simulink model "Dual_EV_Charger_baseline"  (R2025b)
settings: Solver=ode23t  StartTime=0.0  StopTime=0.5  RelTol=1e-3
libraries: fl_lib x98, nesl_utility x24, ee_lib x6, slpidlib x4, batteryecm_lib x4, eePwmGenerator x2
(part 3 of 3)

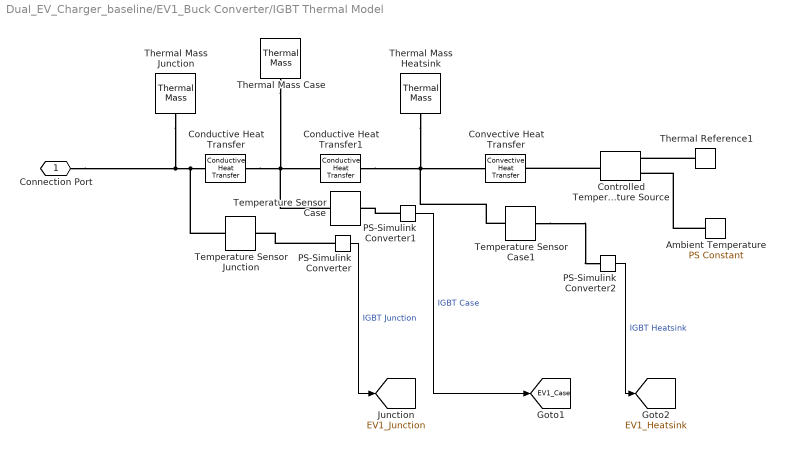
== system Dual_EV_Charger_baseline/EV1_Buck Converter/IGBT Thermal Model ==
  Ambient Temperature : fl_lib/Physical Signals/Sources/PS Constant  constant=298.15
  Conductive Heat Transfer : fl_lib/Thermal/Thermal Elements/Conductive Heat Transfer  thermal_type=foundation.enum.ConstantVariableTabulated.Constant  wall_geometry=foundation.enum.ConductionWallGeometry.Planar  area=5 m^2  thickness=360 m  d_in=0.05 m  d_out=0.1 m  L=1 m  th_cond_min=10 W/(K*m)  th_cond=150 W/(K*m)  th_cond_TLU=[413, 401, 392, 383, 371, 357, 342] W/(K*m)  temp_TLU=[200, 273, 400, 600, 800, 1000, 1200] K  T_specify=off  T_priority=None  T=0 K  T_nominal_specify=off  T_nominal_value=1  T_nominal_unit=K  Q_specify=off  Q_priority=None  Q=0 W  Q_nominal_specify=off  Q_nominal_value=1  Q_nominal_unit=W
  Conductive Heat Transfer1 : fl_lib/Thermal/Thermal Elements/Conductive Heat Transfer  thermal_type=foundation.enum.ConstantVariableTabulated.Constant  wall_geometry=foundation.enum.ConductionWallGeometry.Planar  area=14 m^2  thickness=0.1 m  d_in=0.05 m  d_out=0.1 m  L=1 m  th_cond_min=10 W/(K*m)  th_cond=3 W/(K*m)  th_cond_TLU=[413, 401, 392, 383, 371, 357, 342] W/(K*m)  temp_TLU=[200, 273, 400, 600, 800, 1000, 1200] K  T_specify=off  T_priority=None  T=0 K  T_nominal_specify=off  T_nominal_value=1  T_nominal_unit=K  Q_specify=off  Q_priority=None  Q=0 W  Q_nominal_specify=off  Q_nominal_value=1  Q_nominal_unit=W
  Controlled Temperature Source : fl_lib/Thermal/Thermal Sources/Controlled Temperature Source
  Convective Heat Transfer : fl_lib/Thermal/Thermal Elements/Convective Heat Transfer  thermal_type=foundation.enum.constant_variable.constant  area=40 m^2  heat_tr_coeff=20 W/(K*m^2)  min_heat_tr_coeff=1e-3 W/(K*m^2)  T_specify=off  T_priority=None  T=0 K  T_nominal_specify=off  T_nominal_value=1  T_nominal_unit=K  Q_specify=off  Q_priority=None  Q=0 W  Q_nominal_specify=off  Q_nominal_value=1  Q_nominal_unit=W
  PS-Simulink Converter : nesl_utility/PS-Simulink Converter  PhysicalDomain=network_engine_domain  SubClassName=ps_output  LeftPortType=input  RightPortType=output  PseudoPeriodic=off  Frequencies=[]  VectorFormat=inherit  Unit=inherit  AffineConversion=off
  PS-Simulink Converter1 : nesl_utility/PS-Simulink Converter  PhysicalDomain=network_engine_domain  SubClassName=ps_output  LeftPortType=input  RightPortType=output  PseudoPeriodic=off  Frequencies=[]  VectorFormat=inherit  Unit=inherit  AffineConversion=off
  PS-Simulink Converter2 : nesl_utility/PS-Simulink Converter  PhysicalDomain=network_engine_domain  SubClassName=ps_output  LeftPortType=input  RightPortType=output  PseudoPeriodic=off  Frequencies=[]  VectorFormat=inherit  Unit=inherit  AffineConversion=off
  Temperature Sensor Case : fl_lib/Thermal/Thermal Sensors/Temperature Sensor  temperature_measure=foundation.enum.MeasurementReference.absolute
      settings: InternalSimscapePortConfiguration="{\"Bottom\":[],\"Left\":[{\"id\":\"A\",\"label\":\"A\",\"type\":\"foundation.thermal.thermal\"}],\"Right\":[{\"id\":\"T\",\"label\":\"T\",\"type\":\"output\"}],\"Top\":[]}"
  Temperature Sensor Case1 : fl_lib/Thermal/Thermal Sensors/Temperature Sensor  temperature_measure=foundation.enum.MeasurementReference.absolute
      settings: InternalSimscapePortConfiguration="{\"Bottom\":[],\"Left\":[{\"id\":\"A\",\"label\":\"A\",\"type\":\"foundation.thermal.thermal\"}],\"Right\":[{\"id\":\"T\",\"label\":\"T\",\"type\":\"output\"}],\"Top\":[]}"
  Temperature Sensor Junction : fl_lib/Thermal/Thermal Sensors/Temperature Sensor  temperature_measure=foundation.enum.MeasurementReference.absolute
      settings: InternalSimscapePortConfiguration="{\"Bottom\":[],\"Left\":[{\"id\":\"A\",\"label\":\"A\",\"type\":\"foundation.thermal.thermal\"}],\"Right\":[{\"id\":\"T\",\"label\":\"T\",\"type\":\"output\"}],\"Top\":[]}"
  Thermal Mass Case : fl_lib/Thermal/Thermal Elements/Thermal Mass  mass_type=foundation.enum.constant_variable.constant  mass=0.02 kg  sp_heat=385 J/(K*kg)  mass_min=1e-6 kg  num_ports=foundation.enum.numPorts2.one  m_specify=off  m_priority=High  m=1 kg  m_nominal_specify=off  m_nominal_value=1  m_nominal_unit=kg  T_specify=on  T_priority=High  T=298.15 K  T_nominal_specify=off  T_nominal_value=1  T_nominal_unit=K  Q_specify=off  Q_priority=None  Q=0 W  Q_nominal_specify=off  Q_nominal_value=1  Q_nominal_unit=W
  Thermal Mass Heatsink : fl_lib/Thermal/Thermal Elements/Thermal Mass  mass_type=foundation.enum.constant_variable.constant  mass=0.2 kg  sp_heat=900 J/(K*kg)  mass_min=1e-6 kg  num_ports=foundation.enum.numPorts2.one  m_specify=off  m_priority=High  m=1 kg  m_nominal_specify=off  m_nominal_value=1  m_nominal_unit=kg  T_specify=on  T_priority=High  T=298.15 K  T_nominal_specify=off  T_nominal_value=1  T_nominal_unit=K  Q_specify=off  Q_priority=None  Q=0 W  Q_nominal_specify=off  Q_nominal_value=1  Q_nominal_unit=W
  Thermal Mass Junction : fl_lib/Thermal/Thermal Elements/Thermal Mass  mass_type=foundation.enum.constant_variable.constant  mass=0.001 kg  sp_heat=700 J/(K*kg)  mass_min=1e-6 kg  num_ports=foundation.enum.numPorts2.one  m_specify=off  m_priority=High  m=1 kg  m_nominal_specify=off  m_nominal_value=1  m_nominal_unit=kg  T_specify=on  T_priority=High  T="298.15  K"  T_nominal_specify=off  T_nominal_value=1  T_nominal_unit=K  Q_specify=off  Q_priority=None  Q=0 W  Q_nominal_specify=off  Q_nominal_value=1  Q_nominal_unit=W
  Thermal Reference1 : fl_lib/Thermal/Thermal Elements/Thermal Reference
  Connection Port : PMIOPort  Side=Left
  tag scope: EV1_Case=global, EV1_Heatsink=global, EV1_Junction=global
  wires:
  PS-Simulink Converter/1 -> [EV1_Junction]  "IGBT Junction"
  PS-Simulink Converter1/1 -> [EV1_Case]  "IGBT Case"
  PS-Simulink Converter2/1 -> [EV1_Heatsink]  "IGBT Heatsink"
  connections:
  Conductive Heat Transfer1/RConn1 -- Temperature Sensor Case1/LConn1 -- Thermal Mass Heatsink/LConn1 -- Convective Heat Transfer/LConn1
  Conductive Heat Transfer/RConn1 -- Thermal Mass Case/LConn1 -- Temperature Sensor Case/LConn1 -- Conductive Heat Transfer1/LConn1
  Connection Port/RConn1 -- Thermal Mass Junction/LConn1 -- Temperature Sensor Junction/LConn1 -- Conductive Heat Transfer/LConn1
  Controlled Temperature Source/LConn1 -- Convective Heat Transfer/RConn1
  Thermal Reference1/LConn1 -- Controlled Temperature Source/RConn2
  PS-Simulink Converter/LConn1 -- Temperature Sensor Junction/RConn1
  Ambient Temperature/RConn1 -- Controlled Temperature Source/RConn1
  PS-Simulink Converter1/LConn1 -- Temperature Sensor Case/RConn1
  Temperature Sensor Case1/RConn1 -- PS-Simulink Converter2/LConn1

== system Dual_EV_Charger_baseline/EV1_Plant//EV Battery/EV Battery Thermal Model ==
  Ambient Temperature1 : fl_lib/Physical Signals/Sources/PS Constant  constant=292.15
  Controlled Temperature Source : fl_lib/Thermal/Thermal Sources/Controlled Temperature Source
  Convective Heat Transfer : fl_lib/Thermal/Thermal Elements/Convective Heat Transfer  thermal_type=foundation.enum.constant_variable.constant  area=1e-4 m^2  heat_tr_coeff=20 W/(K*m^2)  min_heat_tr_coeff=1e-3 W/(K*m^2)  T_specify=off  T_priority=None  T=0 K  T_nominal_specify=off  T_nominal_value=1  T_nominal_unit=K  Q_specify=off  Q_priority=None  Q=0 W  Q_nominal_specify=off  Q_nominal_value=1  Q_nominal_unit=W
  PS-Simulink Converter : nesl_utility/PS-Simulink Converter  PhysicalDomain=network_engine_domain  SubClassName=ps_output  LeftPortType=input  RightPortType=output  PseudoPeriodic=off  Frequencies=[]  VectorFormat=inherit  Unit=inherit  AffineConversion=off
  Temperature Sensor : fl_lib/Thermal/Thermal Sensors/Temperature Sensor  temperature_measure=foundation.enum.MeasurementReference.difference
  Thermal Reference : fl_lib/Thermal/Thermal Elements/Thermal Reference
  Thermal Port : PMIOPort  Side=Left
  tag scope: EV1_Tempertaure=global
  wires:
  PS-Simulink Converter/1 -> [EV1_Tempertaure]
  connections:
  Temperature Sensor/LConn1 -- Thermal Port/RConn1 -- Convective Heat Transfer/LConn1
  Convective Heat Transfer/RConn1 -- Controlled Temperature Source/LConn1
  Temperature Sensor/RConn1 -- Controlled Temperature Source/RConn2 -- Thermal Reference/LConn1
  Controlled Temperature Source/RConn1 -- Ambient Temperature1/RConn1
  PS-Simulink Converter/LConn1 -- Temperature Sensor/RConn2

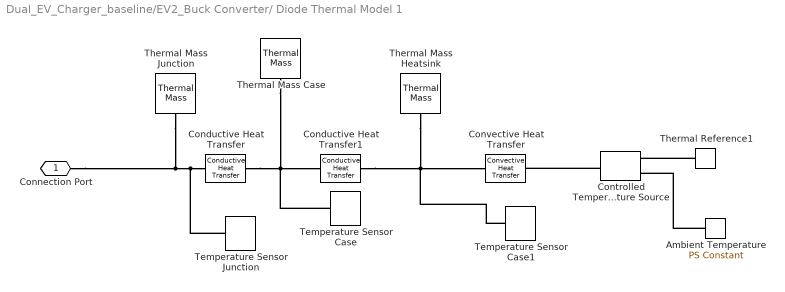
== system Dual_EV_Charger_baseline/EV2_Buck Converter/ Diode Thermal Model 1 ==
  Ambient Temperature : fl_lib/Physical Signals/Sources/PS Constant  constant=298.15
  Conductive Heat Transfer : fl_lib/Thermal/Thermal Elements/Conductive Heat Transfer  thermal_type=foundation.enum.ConstantVariableTabulated.Constant  wall_geometry=foundation.enum.ConductionWallGeometry.Planar  area=5 m^2  thickness=360 m  d_in=0.05 m  d_out=0.1 m  L=1 m  th_cond_min=10 W/(K*m)  th_cond=150 W/(K*m)  th_cond_TLU=[413, 401, 392, 383, 371, 357, 342] W/(K*m)  temp_TLU=[200, 273, 400, 600, 800, 1000, 1200] K  T_specify=off  T_priority=None  T=0 K  T_nominal_specify=off  T_nominal_value=1  T_nominal_unit=K  Q_specify=off  Q_priority=None  Q=0 W  Q_nominal_specify=off  Q_nominal_value=1  Q_nominal_unit=W
  Conductive Heat Transfer1 : fl_lib/Thermal/Thermal Elements/Conductive Heat Transfer  thermal_type=foundation.enum.ConstantVariableTabulated.Constant  wall_geometry=foundation.enum.ConductionWallGeometry.Planar  area=14 m^2  thickness=0.1 m  d_in=0.05 m  d_out=0.1 m  L=1 m  th_cond_min=10 W/(K*m)  th_cond=3 W/(K*m)  th_cond_TLU=[413, 401, 392, 383, 371, 357, 342] W/(K*m)  temp_TLU=[200, 273, 400, 600, 800, 1000, 1200] K  T_specify=off  T_priority=None  T=0 K  T_nominal_specify=off  T_nominal_value=1  T_nominal_unit=K  Q_specify=off  Q_priority=None  Q=0 W  Q_nominal_specify=off  Q_nominal_value=1  Q_nominal_unit=W
  Controlled Temperature Source : fl_lib/Thermal/Thermal Sources/Controlled Temperature Source
  Convective Heat Transfer : fl_lib/Thermal/Thermal Elements/Convective Heat Transfer  thermal_type=foundation.enum.constant_variable.constant  area=40 m^2  heat_tr_coeff=20 W/(K*m^2)  min_heat_tr_coeff=1e-3 W/(K*m^2)  T_specify=off  T_priority=None  T=0 K  T_nominal_specify=off  T_nominal_value=1  T_nominal_unit=K  Q_specify=off  Q_priority=None  Q=0 W  Q_nominal_specify=off  Q_nominal_value=1  Q_nominal_unit=W
  Temperature Sensor Case : fl_lib/Thermal/Thermal Sensors/Temperature Sensor  temperature_measure=foundation.enum.MeasurementReference.absolute
      settings: InternalSimscapePortConfiguration="{\"Bottom\":[],\"Left\":[{\"id\":\"A\",\"label\":\"A\",\"type\":\"foundation.thermal.thermal\"}],\"Right\":[{\"id\":\"T\",\"label\":\"T\",\"type\":\"output\"}],\"Top\":[]}"
  Temperature Sensor Case1 : fl_lib/Thermal/Thermal Sensors/Temperature Sensor  temperature_measure=foundation.enum.MeasurementReference.absolute
      settings: InternalSimscapePortConfiguration="{\"Bottom\":[],\"Left\":[{\"id\":\"A\",\"label\":\"A\",\"type\":\"foundation.thermal.thermal\"}],\"Right\":[{\"id\":\"T\",\"label\":\"T\",\"type\":\"output\"}],\"Top\":[]}"
  Temperature Sensor Junction : fl_lib/Thermal/Thermal Sensors/Temperature Sensor  temperature_measure=foundation.enum.MeasurementReference.absolute
      settings: InternalSimscapePortConfiguration="{\"Bottom\":[],\"Left\":[{\"id\":\"A\",\"label\":\"A\",\"type\":\"foundation.thermal.thermal\"}],\"Right\":[{\"id\":\"T\",\"label\":\"T\",\"type\":\"output\"}],\"Top\":[]}"
  Thermal Mass Case : fl_lib/Thermal/Thermal Elements/Thermal Mass  mass_type=foundation.enum.constant_variable.constant  mass=0.02 kg  sp_heat=385 J/(K*kg)  mass_min=1e-6 kg  num_ports=foundation.enum.numPorts2.one  m_specify=off  m_priority=High  m=1 kg  m_nominal_specify=off  m_nominal_value=1  m_nominal_unit=kg  T_specify=on  T_priority=High  T=298.15 K  T_nominal_specify=off  T_nominal_value=1  T_nominal_unit=K  Q_specify=off  Q_priority=None  Q=0 W  Q_nominal_specify=off  Q_nominal_value=1  Q_nominal_unit=W
  Thermal Mass Heatsink : fl_lib/Thermal/Thermal Elements/Thermal Mass  mass_type=foundation.enum.constant_variable.constant  mass=0.2 kg  sp_heat=900 J/(K*kg)  mass_min=1e-6 kg  num_ports=foundation.enum.numPorts2.one  m_specify=off  m_priority=High  m=1 kg  m_nominal_specify=off  m_nominal_value=1  m_nominal_unit=kg  T_specify=on  T_priority=High  T=298.15 K  T_nominal_specify=off  T_nominal_value=1  T_nominal_unit=K  Q_specify=off  Q_priority=None  Q=0 W  Q_nominal_specify=off  Q_nominal_value=1  Q_nominal_unit=W
  Thermal Mass Junction : fl_lib/Thermal/Thermal Elements/Thermal Mass  mass_type=foundation.enum.constant_variable.constant  mass=0.001 kg  sp_heat=700 J/(K*kg)  mass_min=1e-6 kg  num_ports=foundation.enum.numPorts2.one  m_specify=off  m_priority=High  m=1 kg  m_nominal_specify=off  m_nominal_value=1  m_nominal_unit=kg  T_specify=on  T_priority=High  T="298.15  K"  T_nominal_specify=off  T_nominal_value=1  T_nominal_unit=K  Q_specify=off  Q_priority=None  Q=0 W  Q_nominal_specify=off  Q_nominal_value=1  Q_nominal_unit=W
  Thermal Reference1 : fl_lib/Thermal/Thermal Elements/Thermal Reference
  Connection Port : PMIOPort  Side=Left
  connections:
  Conductive Heat Transfer1/RConn1 -- Thermal Mass Heatsink/LConn1 -- Convective Heat Transfer/LConn1 -- Temperature Sensor Case1/LConn1
  Thermal Mass Case/LConn1 -- Conductive Heat Transfer/RConn1 -- Conductive Heat Transfer1/LConn1 -- Temperature Sensor Case/LConn1
  Thermal Mass Junction/LConn1 -- Temperature Sensor Junction/LConn1 -- Conductive Heat Transfer/LConn1 -- Connection Port/RConn1
  Controlled Temperature Source/LConn1 -- Convective Heat Transfer/RConn1
  Thermal Reference1/LConn1 -- Controlled Temperature Source/RConn2
  Ambient Temperature/RConn1 -- Controlled Temperature Source/RConn1

== system Dual_EV_Charger_baseline/EV2_Buck Converter/ Diode Thermal Model 2 ==
  Ambient Temperature : fl_lib/Physical Signals/Sources/PS Constant  constant=298.15
  Conductive Heat Transfer : fl_lib/Thermal/Thermal Elements/Conductive Heat Transfer  thermal_type=foundation.enum.ConstantVariableTabulated.Constant  wall_geometry=foundation.enum.ConductionWallGeometry.Planar  area=5 m^2  thickness=360 m  d_in=0.05 m  d_out=0.1 m  L=1 m  th_cond_min=10 W/(K*m)  th_cond=150 W/(K*m)  th_cond_TLU=[413, 401, 392, 383, 371, 357, 342] W/(K*m)  temp_TLU=[200, 273, 400, 600, 800, 1000, 1200] K  T_specify=off  T_priority=None  T=0 K  T_nominal_specify=off  T_nominal_value=1  T_nominal_unit=K  Q_specify=off  Q_priority=None  Q=0 W  Q_nominal_specify=off  Q_nominal_value=1  Q_nominal_unit=W
  Conductive Heat Transfer1 : fl_lib/Thermal/Thermal Elements/Conductive Heat Transfer  thermal_type=foundation.enum.ConstantVariableTabulated.Constant  wall_geometry=foundation.enum.ConductionWallGeometry.Planar  area=14 m^2  thickness=0.1 m  d_in=0.05 m  d_out=0.1 m  L=1 m  th_cond_min=10 W/(K*m)  th_cond=3 W/(K*m)  th_cond_TLU=[413, 401, 392, 383, 371, 357, 342] W/(K*m)  temp_TLU=[200, 273, 400, 600, 800, 1000, 1200] K  T_specify=off  T_priority=None  T=0 K  T_nominal_specify=off  T_nominal_value=1  T_nominal_unit=K  Q_specify=off  Q_priority=None  Q=0 W  Q_nominal_specify=off  Q_nominal_value=1  Q_nominal_unit=W
  Controlled Temperature Source : fl_lib/Thermal/Thermal Sources/Controlled Temperature Source
  Convective Heat Transfer : fl_lib/Thermal/Thermal Elements/Convective Heat Transfer  thermal_type=foundation.enum.constant_variable.constant  area=40 m^2  heat_tr_coeff=20 W/(K*m^2)  min_heat_tr_coeff=1e-3 W/(K*m^2)  T_specify=off  T_priority=None  T=0 K  T_nominal_specify=off  T_nominal_value=1  T_nominal_unit=K  Q_specify=off  Q_priority=None  Q=0 W  Q_nominal_specify=off  Q_nominal_value=1  Q_nominal_unit=W
  EV2_Temperature Sensor Case : fl_lib/Thermal/Thermal Sensors/Temperature Sensor  temperature_measure=foundation.enum.MeasurementReference.absolute
      settings: InternalSimscapePortConfiguration="{\"Bottom\":[],\"Left\":[{\"id\":\"A\",\"label\":\"A\",\"type\":\"foundation.thermal.thermal\"}],\"Right\":[{\"id\":\"T\",\"label\":\"T\",\"type\":\"output\"}],\"Top\":[]}"
  EV2_Temperature Sensor Case1 : fl_lib/Thermal/Thermal Sensors/Temperature Sensor  temperature_measure=foundation.enum.MeasurementReference.absolute
      settings: InternalSimscapePortConfiguration="{\"Bottom\":[],\"Left\":[{\"id\":\"A\",\"label\":\"A\",\"type\":\"foundation.thermal.thermal\"}],\"Right\":[{\"id\":\"T\",\"label\":\"T\",\"type\":\"output\"}],\"Top\":[]}"
  EV2_Temperature Sensor Junction : fl_lib/Thermal/Thermal Sensors/Temperature Sensor  temperature_measure=foundation.enum.MeasurementReference.absolute
      settings: InternalSimscapePortConfiguration="{\"Bottom\":[],\"Left\":[{\"id\":\"A\",\"label\":\"A\",\"type\":\"foundation.thermal.thermal\"}],\"Right\":[{\"id\":\"T\",\"label\":\"T\",\"type\":\"output\"}],\"Top\":[]}"
  Thermal Mass Case : fl_lib/Thermal/Thermal Elements/Thermal Mass  mass_type=foundation.enum.constant_variable.constant  mass=0.02 kg  sp_heat=385 J/(K*kg)  mass_min=1e-6 kg  num_ports=foundation.enum.numPorts2.one  m_specify=off  m_priority=High  m=1 kg  m_nominal_specify=off  m_nominal_value=1  m_nominal_unit=kg  T_specify=on  T_priority=High  T=298.15 K  T_nominal_specify=off  T_nominal_value=1  T_nominal_unit=K  Q_specify=off  Q_priority=None  Q=0 W  Q_nominal_specify=off  Q_nominal_value=1  Q_nominal_unit=W
  Thermal Mass Heatsink : fl_lib/Thermal/Thermal Elements/Thermal Mass  mass_type=foundation.enum.constant_variable.constant  mass=0.2 kg  sp_heat=900 J/(K*kg)  mass_min=1e-6 kg  num_ports=foundation.enum.numPorts2.one  m_specify=off  m_priority=High  m=1 kg  m_nominal_specify=off  m_nominal_value=1  m_nominal_unit=kg  T_specify=on  T_priority=High  T=298.15 K  T_nominal_specify=off  T_nominal_value=1  T_nominal_unit=K  Q_specify=off  Q_priority=None  Q=0 W  Q_nominal_specify=off  Q_nominal_value=1  Q_nominal_unit=W
  Thermal Mass Junction : fl_lib/Thermal/Thermal Elements/Thermal Mass  mass_type=foundation.enum.constant_variable.constant  mass=0.001 kg  sp_heat=700 J/(K*kg)  mass_min=1e-6 kg  num_ports=foundation.enum.numPorts2.one  m_specify=off  m_priority=High  m=1 kg  m_nominal_specify=off  m_nominal_value=1  m_nominal_unit=kg  T_specify=on  T_priority=High  T="298.15  K"  T_nominal_specify=off  T_nominal_value=1  T_nominal_unit=K  Q_specify=off  Q_priority=None  Q=0 W  Q_nominal_specify=off  Q_nominal_value=1  Q_nominal_unit=W
  Thermal Reference1 : fl_lib/Thermal/Thermal Elements/Thermal Reference
  Connection Port : PMIOPort  Side=Left
  connections:
  Conductive Heat Transfer1/RConn1 -- Thermal Mass Heatsink/LConn1 -- Convective Heat Transfer/LConn1 -- EV2_Temperature Sensor Case1/LConn1
  Thermal Mass Case/LConn1 -- Conductive Heat Transfer/RConn1 -- Conductive Heat Transfer1/LConn1 -- EV2_Temperature Sensor Case/LConn1
  Thermal Mass Junction/LConn1 -- EV2_Temperature Sensor Junction/LConn1 -- Conductive Heat Transfer/LConn1 -- Connection Port/RConn1
  Controlled Temperature Source/LConn1 -- Convective Heat Transfer/RConn1
  Thermal Reference1/LConn1 -- Controlled Temperature Source/RConn2
  Ambient Temperature/RConn1 -- Controlled Temperature Source/RConn1

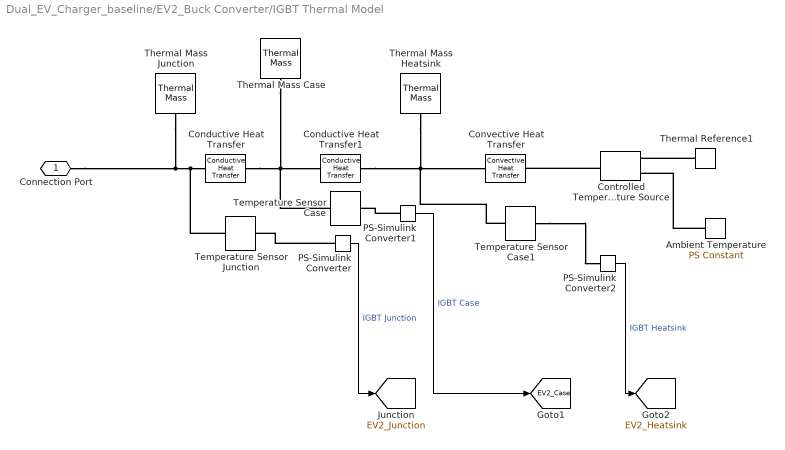
== system Dual_EV_Charger_baseline/EV2_Buck Converter/IGBT Thermal Model ==
  Ambient Temperature : fl_lib/Physical Signals/Sources/PS Constant  constant=298.15
  Conductive Heat Transfer : fl_lib/Thermal/Thermal Elements/Conductive Heat Transfer  thermal_type=foundation.enum.ConstantVariableTabulated.Constant  wall_geometry=foundation.enum.ConductionWallGeometry.Planar  area=5 m^2  thickness=360 m  d_in=0.05 m  d_out=0.1 m  L=1 m  th_cond_min=10 W/(K*m)  th_cond=150 W/(K*m)  th_cond_TLU=[413, 401, 392, 383, 371, 357, 342] W/(K*m)  temp_TLU=[200, 273, 400, 600, 800, 1000, 1200] K  T_specify=off  T_priority=None  T=0 K  T_nominal_specify=off  T_nominal_value=1  T_nominal_unit=K  Q_specify=off  Q_priority=None  Q=0 W  Q_nominal_specify=off  Q_nominal_value=1  Q_nominal_unit=W
  Conductive Heat Transfer1 : fl_lib/Thermal/Thermal Elements/Conductive Heat Transfer  thermal_type=foundation.enum.ConstantVariableTabulated.Constant  wall_geometry=foundation.enum.ConductionWallGeometry.Planar  area=14 m^2  thickness=0.1 m  d_in=0.05 m  d_out=0.1 m  L=1 m  th_cond_min=10 W/(K*m)  th_cond=3 W/(K*m)  th_cond_TLU=[413, 401, 392, 383, 371, 357, 342] W/(K*m)  temp_TLU=[200, 273, 400, 600, 800, 1000, 1200] K  T_specify=off  T_priority=None  T=0 K  T_nominal_specify=off  T_nominal_value=1  T_nominal_unit=K  Q_specify=off  Q_priority=None  Q=0 W  Q_nominal_specify=off  Q_nominal_value=1  Q_nominal_unit=W
  Controlled Temperature Source : fl_lib/Thermal/Thermal Sources/Controlled Temperature Source
  Convective Heat Transfer : fl_lib/Thermal/Thermal Elements/Convective Heat Transfer  thermal_type=foundation.enum.constant_variable.constant  area=40 m^2  heat_tr_coeff=20 W/(K*m^2)  min_heat_tr_coeff=1e-3 W/(K*m^2)  T_specify=off  T_priority=None  T=0 K  T_nominal_specify=off  T_nominal_value=1  T_nominal_unit=K  Q_specify=off  Q_priority=None  Q=0 W  Q_nominal_specify=off  Q_nominal_value=1  Q_nominal_unit=W
  PS-Simulink Converter : nesl_utility/PS-Simulink Converter  PhysicalDomain=network_engine_domain  SubClassName=ps_output  LeftPortType=input  RightPortType=output  PseudoPeriodic=off  Frequencies=[]  VectorFormat=inherit  Unit=inherit  AffineConversion=off
  PS-Simulink Converter1 : nesl_utility/PS-Simulink Converter  PhysicalDomain=network_engine_domain  SubClassName=ps_output  LeftPortType=input  RightPortType=output  PseudoPeriodic=off  Frequencies=[]  VectorFormat=inherit  Unit=inherit  AffineConversion=off
  PS-Simulink Converter2 : nesl_utility/PS-Simulink Converter  PhysicalDomain=network_engine_domain  SubClassName=ps_output  LeftPortType=input  RightPortType=output  PseudoPeriodic=off  Frequencies=[]  VectorFormat=inherit  Unit=inherit  AffineConversion=off
  Temperature Sensor Case : fl_lib/Thermal/Thermal Sensors/Temperature Sensor  temperature_measure=foundation.enum.MeasurementReference.absolute
      settings: InternalSimscapePortConfiguration="{\"Bottom\":[],\"Left\":[{\"id\":\"A\",\"label\":\"A\",\"type\":\"foundation.thermal.thermal\"}],\"Right\":[{\"id\":\"T\",\"label\":\"T\",\"type\":\"output\"}],\"Top\":[]}"
  Temperature Sensor Case1 : fl_lib/Thermal/Thermal Sensors/Temperature Sensor  temperature_measure=foundation.enum.MeasurementReference.absolute
      settings: InternalSimscapePortConfiguration="{\"Bottom\":[],\"Left\":[{\"id\":\"A\",\"label\":\"A\",\"type\":\"foundation.thermal.thermal\"}],\"Right\":[{\"id\":\"T\",\"label\":\"T\",\"type\":\"output\"}],\"Top\":[]}"
  Temperature Sensor Junction : fl_lib/Thermal/Thermal Sensors/Temperature Sensor  temperature_measure=foundation.enum.MeasurementReference.absolute
      settings: InternalSimscapePortConfiguration="{\"Bottom\":[],\"Left\":[{\"id\":\"A\",\"label\":\"A\",\"type\":\"foundation.thermal.thermal\"}],\"Right\":[{\"id\":\"T\",\"label\":\"T\",\"type\":\"output\"}],\"Top\":[]}"
  Thermal Mass Case : fl_lib/Thermal/Thermal Elements/Thermal Mass  mass_type=foundation.enum.constant_variable.constant  mass=0.02 kg  sp_heat=385 J/(K*kg)  mass_min=1e-6 kg  num_ports=foundation.enum.numPorts2.one  m_specify=off  m_priority=High  m=1 kg  m_nominal_specify=off  m_nominal_value=1  m_nominal_unit=kg  T_specify=on  T_priority=High  T=298.15 K  T_nominal_specify=off  T_nominal_value=1  T_nominal_unit=K  Q_specify=off  Q_priority=None  Q=0 W  Q_nominal_specify=off  Q_nominal_value=1  Q_nominal_unit=W
  Thermal Mass Heatsink : fl_lib/Thermal/Thermal Elements/Thermal Mass  mass_type=foundation.enum.constant_variable.constant  mass=0.2 kg  sp_heat=900 J/(K*kg)  mass_min=1e-6 kg  num_ports=foundation.enum.numPorts2.one  m_specify=off  m_priority=High  m=1 kg  m_nominal_specify=off  m_nominal_value=1  m_nominal_unit=kg  T_specify=on  T_priority=High  T=298.15 K  T_nominal_specify=off  T_nominal_value=1  T_nominal_unit=K  Q_specify=off  Q_priority=None  Q=0 W  Q_nominal_specify=off  Q_nominal_value=1  Q_nominal_unit=W
  Thermal Mass Junction : fl_lib/Thermal/Thermal Elements/Thermal Mass  mass_type=foundation.enum.constant_variable.constant  mass=0.001 kg  sp_heat=700 J/(K*kg)  mass_min=1e-6 kg  num_ports=foundation.enum.numPorts2.one  m_specify=off  m_priority=High  m=1 kg  m_nominal_specify=off  m_nominal_value=1  m_nominal_unit=kg  T_specify=on  T_priority=High  T="298.15  K"  T_nominal_specify=off  T_nominal_value=1  T_nominal_unit=K  Q_specify=off  Q_priority=None  Q=0 W  Q_nominal_specify=off  Q_nominal_value=1  Q_nominal_unit=W
  Thermal Reference1 : fl_lib/Thermal/Thermal Elements/Thermal Reference
  Connection Port : PMIOPort  Side=Left
  tag scope: EV2_Case=global, EV2_Heatsink=global, EV2_Junction=global
  wires:
  PS-Simulink Converter/1 -> [EV2_Junction]  "IGBT Junction"
  PS-Simulink Converter1/1 -> [EV2_Case]  "IGBT Case"
  PS-Simulink Converter2/1 -> [EV2_Heatsink]  "IGBT Heatsink"
  connections:
  Conductive Heat Transfer1/RConn1 -- Temperature Sensor Case1/LConn1 -- Thermal Mass Heatsink/LConn1 -- Convective Heat Transfer/LConn1
  Conductive Heat Transfer/RConn1 -- Thermal Mass Case/LConn1 -- Temperature Sensor Case/LConn1 -- Conductive Heat Transfer1/LConn1
  Connection Port/RConn1 -- Thermal Mass Junction/LConn1 -- Temperature Sensor Junction/LConn1 -- Conductive Heat Transfer/LConn1
  Controlled Temperature Source/LConn1 -- Convective Heat Transfer/RConn1
  Thermal Reference1/LConn1 -- Controlled Temperature Source/RConn2
  PS-Simulink Converter/LConn1 -- Temperature Sensor Junction/RConn1
  Ambient Temperature/RConn1 -- Controlled Temperature Source/RConn1
  PS-Simulink Converter1/LConn1 -- Temperature Sensor Case/RConn1
  Temperature Sensor Case1/RConn1 -- PS-Simulink Converter2/LConn1

== system Dual_EV_Charger_baseline/EV2_Plant//EV Battery1/EV Battery Thermal Model ==
  Ambient Temperature1 : fl_lib/Physical Signals/Sources/PS Constant  constant=292.15
  Controlled Temperature Source : fl_lib/Thermal/Thermal Sources/Controlled Temperature Source
  Convective Heat Transfer : fl_lib/Thermal/Thermal Elements/Convective Heat Transfer  thermal_type=foundation.enum.constant_variable.constant  area=1e-4 m^2  heat_tr_coeff=20 W/(K*m^2)  min_heat_tr_coeff=1e-3 W/(K*m^2)  T_specify=off  T_priority=None  T=0 K  T_nominal_specify=off  T_nominal_value=1  T_nominal_unit=K  Q_specify=off  Q_priority=None  Q=0 W  Q_nominal_specify=off  Q_nominal_value=1  Q_nominal_unit=W
  PS-Simulink Converter : nesl_utility/PS-Simulink Converter  PhysicalDomain=network_engine_domain  SubClassName=ps_output  LeftPortType=input  RightPortType=output  PseudoPeriodic=off  Frequencies=[]  VectorFormat=inherit  Unit=inherit  AffineConversion=off
  Temperature Sensor : fl_lib/Thermal/Thermal Sensors/Temperature Sensor  temperature_measure=foundation.enum.MeasurementReference.difference
  Thermal Reference : fl_lib/Thermal/Thermal Elements/Thermal Reference
  Thermal Port : PMIOPort  Side=Left
  tag scope: EV2_Tempertaure=global
  wires:
  PS-Simulink Converter/1 -> [EV2_Tempertaure]
  connections:
  Temperature Sensor/LConn1 -- Thermal Port/RConn1 -- Convective Heat Transfer/LConn1
  Convective Heat Transfer/RConn1 -- Controlled Temperature Source/LConn1
  Temperature Sensor/RConn1 -- Controlled Temperature Source/RConn2 -- Thermal Reference/LConn1
  Controlled Temperature Source/RConn1 -- Ambient Temperature1/RConn1
  PS-Simulink Converter/LConn1 -- Temperature Sensor/RConn2

== system Dual_EV_Charger_baseline/Input Measurements & Analysis/SOC Coulomb Counting ==
  socOutCell : Inport
  Constant2 : Constant  Value=6.28
  Constant3 : Constant  Value=3600
  Divide : Product  Inputs=*/
  Gain : Gain  Gain=100
  Product : Product
  Out1 : Outport
  wires:
  Constant3/1 -> Product/1
  Product/1 -> Divide/2
  socOutCell/1 -> Divide/1
  Gain/1 -> Out1/1
  Constant2/1 -> Product/2
  Divide/1 -> Gain/1

== system Dual_EV_Charger_baseline/Input Measurements & Analysis1/SOC Coulomb Counting ==
  socOutCell : Inport
  Constant2 : Constant  Value=6.28
  Constant3 : Constant  Value=3600
  Divide : Product  Inputs=*/
  Gain : Gain  Gain=100
  Product : Product
  Out1 : Outport
  wires:
  Constant3/1 -> Product/1
  Product/1 -> Divide/2
  socOutCell/1 -> Divide/1
  Gain/1 -> Out1/1
  Constant2/1 -> Product/2
  Divide/1 -> Gain/1

== system Dual_EV_Charger_baseline/Output Measurements & Analysis/SOC Coulomb Counting ==
  socOutCell : Inport
  Constant2 : Constant  Value=309
  Constant3 : Constant  Value=3600
  Divide : Product  Inputs=*/
  Gain : Gain  Gain=100
  Product : Product
  Out1 : Outport
  wires:
  Product/1 -> Divide/2
  Constant2/1 -> Product/2
  Constant3/1 -> Product/1
  Gain/1 -> Out1/1
  socOutCell/1 -> Divide/1
  Divide/1 -> Gain/1

== system Dual_EV_Charger_baseline/Output Measurements & Analysis1/SOC Coulomb Counting ==
  socOutCell : Inport
  Constant2 : Constant  Value=309
  Constant3 : Constant  Value=3600
  Divide : Product  Inputs=*/
  Gain : Gain  Gain=100
  Product : Product
  Out1 : Outport
  wires:
  Product/1 -> Divide/2
  Constant2/1 -> Product/2
  Constant3/1 -> Product/1
  Gain/1 -> Out1/1
  socOutCell/1 -> Divide/1
  Divide/1 -> Gain/1

== stateflow chart Dual_EV_Charger_baseline/CC-CV Logic1 ==
  state CC
    during:
    Mode = 0;
  state CV
    during:
    Mode = 1;
  (default) -> CC
  CC -> CV : [Vout >= 294.35]
  data: Vout input; Mode output double

== stateflow chart Dual_EV_Charger_baseline/Current Termination Logic ==
  state Charging
    during:
    Iref_out = Iref_in;
    Charge_Enable = 1;
  state Charge_Finish
    during:
    Charge_Enable = 0;
  (default) -> Charging
  Charging -> Charge_Finish : [Mode == 1 && Icharge <= 30.9]
  data: Iref_out output double size=1; Charge_Enable output; Icharge input; Iref_in input double size=1; Mode input

== stateflow chart Dual_EV_Charger_baseline/CC-CV Logic ==
  state CC
    during:
    Mode = 0;
  state CV
    during:
    Mode = 1;
  (default) -> CC
  CC -> CV : [Vout >= 294.35]
  data: Vout input; Mode output double

== stateflow chart Dual_EV_Charger_baseline/Current Termination Logic1 ==
  state Charging
    during:
    Iref_out = Iref_in;
    Charge_Enable = 1;
  state Charge_Finish
    during:
    Charge_Enable = 0;
  (default) -> Charging
  Charging -> Charge_Finish : [Mode == 1 && Icharge <= 30.9]
  data: Iref_out output double size=1; Charge_Enable output; Icharge input; Iref_in input double size=1; Mode input

== matlab function Dual_EV_Charger_baseline/Charging Efficiency/MATLAB Function ==
  data: Pout input; eta output; Pin input
function eta = calculateEfficiency(Pout, Pin)
%#codegen

if Pin > 1
    eta = 100 * Pout / Pin;
else
    eta = 0;
end

end

== matlab function Dual_EV_Charger_baseline/Charging Efficiency1/MATLAB Function ==
  data: Pout input; eta output; Pin input
function eta = calculateEfficiency(Pout, Pin)
%#codegen

if Pin > 1
    eta = 100 * Pout / Pin;
else
    eta = 0;
end

end
